simulink model "CLLCResonantConverter"  (R2026a)
settings: Solver=ode23t  StopTime=0.018  FixedStep=1e-4  MaxStep=1e-6  AbsTol=1e-3
PreLoadFcn:
  | % Parameterize the model
  | 
  | if ~exist('CLLCDesign', 'var')
  | CLLCConverterDefaultInputParameters;
  | end
undefined symbols (not defined in the file): CLLCController, CLLCDesign
libraries: fl_lib x46, nesl_utility x45, ee_lib x35, ConverterLibrary x1
(part 1 of 4)
Description:
  | Design of LLC Resonant Converter
settings Model: SimulationMode=accelerator  ExtModeTrigDuration=100  Creator=The MathWorks, Inc.  LastModifiedBy=vsolaise
settings SolverCC: MaxConsecutiveMinStep=10
settings DataIOCC: StateSaveName=tmp_raccel_xout  SignalLoggingName=logsoutCLLCConverter  OutputTimes=[0:1.1*3*Voc/(1*2000):1.1*3*Voc/1]
settings OptimizationCC: EfficientMapNaN2IntZero=off
settings HardwareCC: ProdHWDeviceType=Intel->x86-32 (Windows32)  TargetBitPerPointer=64.0  TargetBitPerSizeT=64.0  TargetBitPerPtrDiffT=64.0  TargetLongLongMode=on  TargetIntDivRoundTo=Zero  TargetEndianess=LittleEndian  TargetWordSize=64.0  TargetHWDeviceType=MATLAB Host  ProdEqTarget=off
settings RTWCC: SystemTargetFile=raccel.tlc  TemplateMakefile=raccel_default_tmf  RTWVerbose=off  RTWUseSimCustomCode=on
settings CodeAppCC: GenerateComments=off  MaxIdLength=128.0  SimulinkBlockComments=off
settings RaccelTargetCC: ExtModeTransport=0.0  ExtModeStaticAllocSize=1000000.0  ENABLE_SLEXEC_SSBRIDGE=1.0  RTWCAPIParams=on  RTWCAPIRootIO=on  MultiwordLength=2048.0
settings SimscapeCC: SimscapeNominalValues="[{\"value\":\"1\",\"unit\":\"A\"},{\"value\":\"1\",\"unit\":\"bar\"},{\"value\":\"1\",\"unit\":\"cm^2\"},{\"value\":\"1\",\"unit\":\"cm^3/s\"},{\"value\":\"1\",\"unit\":\"kJ/kg\"},{\"value\":\"1\",\"unit\":\"kW\"},{\"value\":\"1\",\"unit\":\"l\"},{\"value\":\"1\",\"unit\":\"N\"},{\"value\":\"1\",\"unit\":\"N*m\"},{\"value\":\"1\",\"unit\":\"V\"}]"  SimscapeLogName=SimlogCLLCConverter  SimscapeLogLimitData=off  SimscapeLogDataHistory=5000.0

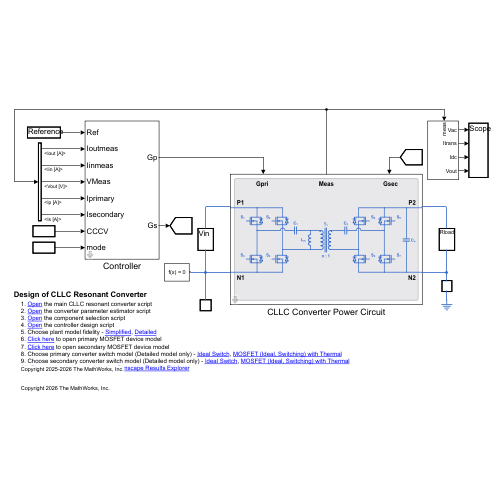
[thumbnail: Simulink's stored preview of the top-level diagram]
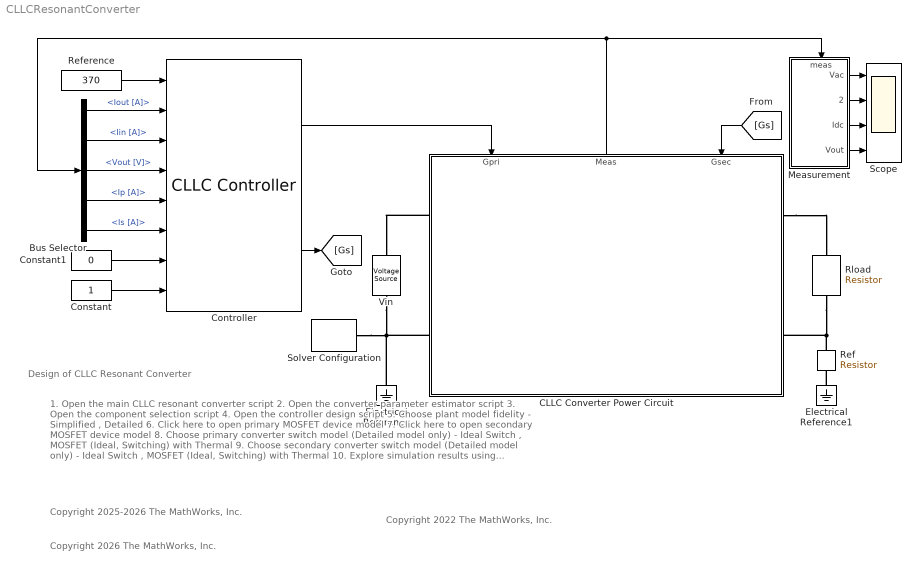
== system CLLCResonantConverter ==
  note: Copyright 2025-2026 The MathWorks, Inc.
  note: 1. Open the main CLLC resonant converter script
      | 2. Open the converter parameter estimator script
      | 3. Open the component selection script
      | 4. Open the controller design script
      | 5. Choose plant model fidelity - Simplified , Detailed
      | 6. Click here to open primary MOSFET device model
      | 7. Click here to open secondary MOSFET device model
      | 8. Choose primary converter switch model (Detailed model only) - Ideal Switch , MOSFET (Ideal, Switching) with Thermal
      | 9. Choose secondary converter switch model (Detailed model only) - Ideal Switch , MOSFET (Ideal, Switching) with Thermal
      | 10. Explore simulation results using Simscape Results Explorer
  note: Design of CLLC Resonant Converter
  note: Copyright 2022 The MathWorks, Inc.
  note: Copyright 2026 The MathWorks, Inc.
  Bus Selector : BusSelector  OutputSignals=Rectifier.Iout [A],Inverter.Iin [A],Rectifier.Vout [V],ResonantTank.Ip [A],ResonantTank.Is [A]
  CLLC Converter Power Circuit : Subsystem  mask(CLLC Converter Plant){modelOption=Simplified, C1=CLLCDesign.C1, C1_unit=F, Rcr1=CLLCDesign.Rcr1, Rcr1_unit=Ohm, C2=CLLCDesign.C2, C2_unit=F, Rcr2=CLLCDesign.Rcr2, Rcr2_unit=Ohm, Llk1=CLLCDesign.Llk1, Llk1_unit=H, R1=CLLCDesign.R1, R1_unit=Ohm, Llk2=CLLCDesign.Llk2, Llk2_unit=H, R2=CLLCDesign.R2, R2_unit=Ohm, Lm=CLLCDesign.Lm, Lm_unit=H, N1=CLLCDesign.N1, N2=CLLCDesign.N2, Co=CLLCDesign.Co, Co_unit=F, Rco=CLLCDesign.Rco, Rco_unit=Ohm, Vco=350, Vco_unit=V, PrimaryDeviceOption=MOSFET (Ideal, Switching) with Thermal, PrimaryRon=0.0001, PrimaryRon_unit=Ohm, PrimaryGoff=1e-5, PrimaryGoff_unit=1/Ohm, PrimaryVth=2.5, PrimaryVth_unit=V, PrimaryVbodydiodeOn=0.6, PrimaryVbodydiodeOn_unit=V, PrimaryRbodydiodeOn=0.0001, PrimaryRbodydiodeOn_unit=Ohm, PrimaryGbodydiodeOff=1e-5, PrimaryGbodydiodeOff_unit=1/Ohm, PrimaryCparasitic=CLLCDesign.Cparasitic, PrimaryCparasitic_unit=F, SecondaryDeviceOption=MOSFET (Ideal, Switching) with Thermal, SecondaryRon=0.0001, SecondaryRon_unit=Ohm, SecondaryGoff=1e-5, SecondaryGoff_unit=1/Ohm, SecondaryVth=2.5, SecondaryVth_unit=V, SecondaryVbodydiodeOn=0.6, SecondaryVbodydiodeOn_unit=V, SecondaryRbodydiodeOn=0.0001, SecondaryRbodydiodeOn_unit=Ohm, SecondaryGbodydiodeOff=1e-5, SecondaryGbodydiodeOff_unit=1/Ohm, SecondaryCparasitic=CLLCDesign.Cparasitic, SecondaryCparasitic_unit=F, PrimarySimTemp=25, PrimarySimTemp_unit=degC, SecondarySimTemp=25, SecondarySimTemp_unit=degC}
      mask prompts: modelOption "Model option"; C1 "Primary resonant capacitance (C1)"; Rcr1 "Primary resonant capacitor ESR (Rcr1)"; C2 "Secondary resonant capacitance (C2)"; Rcr2 "Secondary resonant capacitor ESR (Rcr2)"; Llk1 "Primary leakage inductance (Llk1)"; R1 "Primary resistance (R1)"; Llk2 "Secondary leakage inductance (Llk2)"; R2 "Secondary resistance (R2)"; Lm "Magnetizing inductance (Lm)"; N1 "Transformer primary number of turns (N1)"; N2 "Transformer secondary number of turns (N2)"; Co "Secondary output capacitance (Co)"; Rco "Secondary output capacitance ESR (Rco)"; Vco "Initial output capacitor voltage"; PrimaryDeviceOption "Select the primary switching device"; PrimaryRon "On-state resistance"; PrimaryGoff "Off-state conductance"; PrimaryVth "Threshold voltage"; PrimaryVbodydiodeOn "Body diode forward voltage"; PrimaryRbodydiodeOn "Body diode on-resistance"; PrimaryGbodydiodeOff "Body diode off-conductance"; PrimaryCparasitic "MOSFET parasitic capacitance"; SecondaryDeviceOption "Select the secondary switching device"; SecondaryRon "On-state resistance"; SecondaryGoff "Off-state conductance"; SecondaryVth "Threshold voltage"; SecondaryVbodydiodeOn "Body diode forward voltage"; SecondaryRbodydiodeOn "Body diode on-resistance"; SecondaryGbodydiodeOff "Body diode off-conductance"; SecondaryCparasitic "MOSFET parasitic capacitance"; PrimarySimTemp "Simulation temperature"; SecondarySimTemp "Simulation temperature"
      mask help: This block models the power circuit of the CLLC resonant converter. You can choose between different semicondcutor switch model for primary and secondaryconverter. You can choose between ideal semiconductor switch, MOSFET without thermal port and tabulated MOSFET with thermal port.
      mask init:
      | %% Unit conversion: convert displayed values to base SI units
      | convMap = containers.Map( ...
      |     {'W','kW','MW','V','kV','mV','F','mF','uF','nF','pF', ...
      |      'H','mH','uH','nH','Ohm','kOhm','mOhm','S','mS','1/Ohm'}, ...
      |     {1, 1e3, 1e6, 1, 1e3, 1e-3, 1, 1e-3, 1e-6, 1e-9, 1e-12, ...
      |      1, 1e-3, 1e-6, 1e-9, 1, 1e3, 1e-3, 1, 1e-3, 1});
      | C1 = C1 * convMap(C1_unit);
      | Rcr1 = Rcr1 * convMap(Rcr1_unit);
      | C2 = C2 * convMap(C2_unit);
      | Rcr2 = Rcr2 * convMap(Rcr2_unit);
      | Llk1 = Llk1 * convMap(Llk1_unit);
      | R1 = R1 * convMap(R1_unit);
      | Llk2 = Llk2 * convMap(Llk2_unit);
      | R2 = R2 * convMap(R2_unit);
      | Lm = Lm * convMap(Lm_unit);
      | Co = Co * convMap(Co_unit);
      | Rco = Rco * convMap(Rco_unit);
      | Vco = Vco * convMap(Vco_unit);
      | PrimaryRon = PrimaryRon * convMap(PrimaryRon_unit);
      | PrimaryGoff = PrimaryGoff * convMap(PrimaryGoff_unit);
      | PrimaryVth = PrimaryVth * convMap(PrimaryVth_unit);
      | PrimaryVbodydiodeOn = PrimaryVbodydiodeOn * convMap(PrimaryVbodydiodeOn_unit);
      | PrimaryRbodydiodeOn = PrimaryRbodydiodeOn * convMap(PrimaryRbodydiodeOn_unit);
      | PrimaryGbodydiodeOff = PrimaryGbodydiodeOff * convMap(PrimaryGbodydiodeOff_unit);
      | PrimaryCparasitic = PrimaryCparasitic * convMap(PrimaryCparasitic_unit);
      | SecondaryRon = SecondaryRon * convMap(SecondaryRon_unit);
      | SecondaryGoff = SecondaryGoff * convMap(SecondaryGoff_unit);
      | SecondaryVth = SecondaryVth * convMap(SecondaryVth_unit);
      | SecondaryVbodydiodeOn = SecondaryVbodydiodeOn * convMap(SecondaryVbodydiodeOn_unit);
      | SecondaryRbodydiodeOn = SecondaryRbodydiodeOn * convMap(SecondaryRbodydiodeOn_unit);
      | SecondaryGbodydiodeOff = SecondaryGbodydiodeOff * convMap(SecondaryGbodydiodeOff_unit);
      | SecondaryCparasitic = SecondaryCparasitic * convMap(SecondaryCparasitic_unit);
      | % Simulation temperature (primary bridge, thermal MOSFETs)
      | % Temperature is an OFFSET unit (K = degC + 273.15), so it cannot use the
      | % multiplicative convMap above; convert it explicitly. PrimarySimTemp_K is read directly
      | % by each primary thermal MOSFET junction-temperature initial target and by every
      | % Temperature Source in the primary bridge.
      | if strcmp(PrimarySimTemp_unit, 'degC')
      |     PrimarySimTemp_K = PrimarySimTemp + 273.15;
      | elseif strcmp(PrimarySimTemp_unit, 'K')
      |     PrimarySimTemp_K = PrimarySimTemp;
      | else
      |     error('CLLC Converter Power Circuit: unrecognized simulation-temperature unit "%s" (expected degC or K).', PrimarySimTemp_unit);
      | end
      | % Simulation temperature (secondary bridge, thermal MOSFETs)
      | % Temperature is an OFFSET unit (K = degC + 273.15), so it cannot use the
      | % multiplicative convMap above; convert it explicitly. SecondarySimTemp_K is read directly
      | % by each secondary thermal MOSFET junction-temperature initial target and by every
      | % Temperature Source in the secondary bridge.
      | if strcmp(SecondarySimTemp_unit, 'degC')
      |     SecondarySimTemp_K = SecondarySimTemp + 273.15;
      | elseif strcmp(SecondarySimTemp_unit, 'K')
      |     SecondarySimTemp_K = SecondarySimTemp;
      | else
      |     error('CLLC Converter Power Circuit: unrecognized simulation-temperature unit "%s" (expected degC or K).', SecondarySimTemp_unit);
      | end
      settings: CopyFcn="set_param(gcbh,\"LinkStatus\",\"none\");"  PortSchema="{\"entries\":[{\"content\":{\"sides\":[{\"content\":{\"connectorIds\":[\"LConn1\",\"LConn2\"]},\"type\":\"ConnectorPlacement.EquallySpacedRectSide\",\"uuid\":\"0e984043-8111-4613-9feb-f4d4d19f792a\"},{\"content\":{\"connectorIds\":[\"RConn1\",\"RConn2\"],\"side\":\"RIGHT\"},\"type\":\"ConnectorPlacement.EquallySpacedRectSide\",\"uuid\":\"aee9207a-aaf7-4114-a348-153041cb19a5\"},{\"content\":{\"connectorIds\":[\"In1\",\"Out1\",\"In2\"],\"side\":\"TOP\"},\"type\":\"ConnectorPlacement.EquallySpacedRectSide\",\"uuid\":\"cf17a722-cb18-4642-bf19-4f4ee8ce3a25\"}]},\"type\":\"ConnectorPlacement.EquallySpacedConnector\",\"uuid\":\"0a50e5d5-a4bf-4817-9816-42fb9bad860d\"}],\"packageUris\":[\"http://schema.mathworks.com/mf0/Connector/R2020b\"],\"version\":\"1.0\"}"
      mask Help: web('CLLCPowerCircuit.html')
      mask TypeOptions modelOption: Simplified | Detailed
      mask Callback modelOption: selectCLLCConverterModelOption(gcb);
      mask TypeOptions C1_unit: F | mF | uF | nF | pF
      mask TypeOptions Rcr1_unit: Ohm | kOhm | mOhm
      mask TypeOptions C2_unit: F | mF | uF | nF | pF
      mask TypeOptions Rcr2_unit: Ohm | kOhm | mOhm
      mask TypeOptions Llk1_unit: H | mH | uH | nH
      mask TypeOptions R1_unit: Ohm | kOhm | mOhm
      mask TypeOptions Llk2_unit: H | mH | uH | nH
      mask TypeOptions R2_unit: Ohm | kOhm | mOhm
      mask TypeOptions Lm_unit: H | mH | uH | nH
      mask TypeOptions Co_unit: F | mF | uF | nF | pF
      mask TypeOptions Rco_unit: Ohm | kOhm | mOhm
      mask TypeOptions Vco_unit: V | kV | mV
      mask TypeOptions PrimaryDeviceOption: Ideal Switch | MOSFET (Ideal, Switching) with Thermal
      mask Callback PrimaryDeviceOption: selectCLLCPrimaryMOSFET(gcb);
      mask TypeOptions PrimaryRon_unit: Ohm | kOhm | mOhm
      mask TypeOptions PrimaryGoff_unit: 1/Ohm | S | mS
      mask TypeOptions PrimaryVth_unit: V | kV | mV
      mask TypeOptions PrimaryVbodydiodeOn_unit: V | mV
      mask TypeOptions PrimaryRbodydiodeOn_unit: Ohm | kOhm | mOhm
      mask TypeOptions PrimaryGbodydiodeOff_unit: 1/Ohm | S | mS
      mask TypeOptions PrimaryCparasitic_unit: F | mF | uF | nF | pF
      mask TypeOptions SecondaryDeviceOption: Ideal Switch | MOSFET (Ideal, Switching) with Thermal
      mask Callback SecondaryDeviceOption: selectCLLCSecondaryMOSFET(gcb);
      mask TypeOptions SecondaryRon_unit: Ohm | kOhm | mOhm
      mask TypeOptions SecondaryGoff_unit: 1/Ohm | S | mS
      mask TypeOptions SecondaryVth_unit: V | kV | mV
      mask TypeOptions SecondaryVbodydiodeOn_unit: V | mV
      mask TypeOptions SecondaryRbodydiodeOn_unit: Ohm | kOhm | mOhm
      mask TypeOptions SecondaryGbodydiodeOff_unit: 1/Ohm | S | mS
      mask TypeOptions SecondaryCparasitic_unit: F | mF | uF | nF | pF
      mask TypeOptions PrimarySimTemp_unit: degC | K
      mask TypeOptions SecondarySimTemp_unit: degC | K
      mask DialogControl ParameterGroupVar Prompt: CLLC Resonant Converter Plant
      mask DialogControl CLLCTank Prompt: CLLC converter parameters
      mask DialogControl TransformerParameters Prompt: Transformer
      mask DialogControl PrimarySwitch Prompt: Primary semiconductor switch
      mask DialogControl PrimaryOpenMOSFETMask Prompt: Open the MOSFET block mask
      mask DialogControl PrimaryOpenMOSFETMask Callback: openCLLCDeviceMask(gcb, 'primaryThermalMOSFET');
      mask DialogControl PrimaryApplyMOSFETParam Prompt: Apply parameters to all primary MOSFET blocks
      mask DialogControl PrimaryApplyMOSFETParam Callback: applyCLLCDeviceParameters(gcb, 'primaryThermalMOSFET');
      mask DialogControl SecondarySwitch Prompt: Secondary semiconductor switch
      mask DialogControl SecondaryOpenMOSFETMask Prompt: Open the MOSFET block mask
      mask DialogControl SecondaryOpenMOSFETMask Callback: openCLLCDeviceMask(gcb, 'secondaryThermalMOSFET');
      mask DialogControl SecondaryApplyMOSFETParam Prompt: Apply parameters to all secondary MOSFET blocks
      mask DialogControl SecondaryApplyMOSFETParam Callback: applyCLLCDeviceParameters(gcb, 'secondaryThermalMOSFET');
      mask DialogControl ExportPanel Prompt: Export to Unmasked Subsystem
      mask DialogControl ExportInfo Prompt: To customize the converter, export it as an unmasked subsystem with the active variant flattened - a standalone, fully-editable circuit plus a parameter file. Requires the "Variant Manager for Simulink" add-on.
      mask DialogControl exportToModel Prompt: Export
      mask DialogControl exportToModel Callback: exportConverterModelFromMask(gcb);
      mask Display: image('CLLCConverterIcon.svg');
  Constant : Constant
  Constant1 : Constant  Value=0
  Controller : ConverterLibrary/Controller/Soft-Switching Converters/CLLC Controller  controllerDomain=Continuous  resFreq=CLLCDesign.resonantFreq  ratedPower=CLLCSpec.ratedOutputPower.value  Fmin=CLLCController.minPUfrequency  Fmax=CLLCController.maxPUfrequency  Tdead=CLLCController.deadTime  VdcValue=CLLCSpec.maxInputVoltage.value  Kpv=CLLCController.Kpv  Kiv=CLLCController.Kiv  Kid=0  IdcMax=2.5  IdcMin=-2.5  cntrlSelect=2P2Z compensator  Kc=CLLCCompensator.Ki  numSdomain=CLLCCompensator.numSDomain  denSdomain=CLLCCompensator.denSDomain  numZdomain=CLLCCompensator.numZDomain  denZdomain=CLLCCompensator.denZDomain  Kp=CLLCController.Kp  Ki=CLLCController.Ki  Ith=CLLCCompensator.SRCurrentThreshold  Ibw=300000  vcoSelect=Constant rate  vcoGain=CLLCController.constantVCOGain  vcoGainVec=CLLCController.vcoGainVec  pwmSampleTime=CLLCController.deadTime/2  TsVoltage=CLLCController.TsVoltage  TsCurrent=CLLCController.TsCurrent
      link override 2P2Z Compensator: LabelModeActiveChoice=SCompensator
      link override VCO: LabelModeActiveChoice=Constant
      settings: SourceProductName=Simscape Power Converter Components
  Electrical Reference : fl_lib/Electrical/Electrical Elements/Electrical Reference
  Electrical Reference1 : fl_lib/Electrical/Electrical Elements/Electrical Reference
  Measurement : Subsystem
      settings: PortSchema="{\"entries\":[{\"content\":{\"sides\":[{\"content\":{},\"type\":\"ConnectorPlacement.EquallySpacedRectSide\",\"uuid\":\"b5c92219-bd3b-44a8-8a16-1ea587978409\"},{\"content\":{\"connectorIds\":[\"Out1\",\"Out2\",\"Out3\",\"Out4\"],\"side\":\"RIGHT\"},\"type\":\"ConnectorPlacement.EquallySpacedRectSide\",\"uuid\":\"b58951fa-0a4a-415c-91fc-a01c5851cf7b\"},{\"content\":{\"connectorIds\":[\"In1\"],\"side\":\"TOP\"},\"type\":\"ConnectorPlacement.EquallySpacedRectSide\",\"uuid\":\"5d7f8742-bb02-4261-b191-4137e05aff11\"}]},\"type\":\"ConnectorPlacement.EquallySpacedConnector\",\"uuid\":\"cec0d984-b283-4d36-85e7-6ccc2789e1e2\"}],\"packageUris\":[\"http://schema.mathworks.com/mf0/Connector/R2020b\"],\"version\":\"1.0\"}"
  Ref : fl_lib/Electrical/Electrical Elements/Resistor  R=1e5 Ohm  i_specify=off  i_priority=None  i=0 A  i_nominal_specify=off  i_nominal_value=1  i_nominal_unit=A  v_specify=off  v_priority=None  v=0 V  v_nominal_specify=off  v_nominal_value=1  v_nominal_unit=V
  Reference : Constant  Value=370
  Rload : fl_lib/Electrical/Electrical Elements/Resistor  R=19.55 Ohm  i_specify=off  i_priority=None  i=0 A  i_nominal_specify=off  i_nominal_value=1  i_nominal_unit=A  v_specify=off  v_priority=None  v=0 V  v_nominal_specify=off  v_nominal_value=1  v_nominal_unit=V
  Scope : Scope  NumInputPorts=4
      settings: Title=Resonant Tank Voltages  ActiveDisplayYMinimum=-489.00804394108224  ActiveDisplayYMaximum=489.00846158085653
  Solver Configuration : nesl_utility/Solver Configuration  PhysicalDomain=network_engine_domain  SubClassName=solver  LeftPortType=input  RightPortType=generic  Tones=[]  Harmonics=[]  SimulateNoise=off  Profile=off  UseLocalSampling=off  EnableSwitchedLinearOptims=on  FrequencyDomain=off  UseCCode=off  RelTol=0.001  AbsTol=0.001  MinStep=1e-09  ToWorkspace=off  RevertToSquareIcSolve=off  NumHomotopyIterations=100  PhasorMode=off  PhasorModeNumHarmonics=1  ConsistencySolver=NEWTON_XTOL_AFTER_FTOL  CanonicalOrdering=UNORDERED  OptimizeIntermediates=UNOPTIMIZED  IndexReductionMethod=DerivativeReplacement  DoDC=off  ResidualTolerance=1e-09  ConsistencyTolSource=GLOBAL  ConsistencyAbsTol=0.001  ConsistencyRelTol=0.001  ConsistencyTolFactor=0.001  UseLocalSolver=on  LocalSolverChoice=NE_BACKWARD_EULER_ADVANCER  ResolveIndetEquations=off  FunctionEvalNumThread=1  LocalSolverSampleTime=CLLCController.deadTime/3  DoFixedCost=on  MaxNonlinIter=5  MaxModeIter=10  ComputeImpulses=off  ImpulseIterations=2  LinearAlgebra=auto  LinearAlgebraNumThread=0  EquationFormulation=NE_TIME_EF  DelaysMemoryBudget=1024  AutomaticFiltering=on  FilteringTimeConstant=0.001  PartitionStorageMethod=AS_NEEDED  PartitionMemoryBudget=1024  PartitionMethod=ROBUST  MultibodyUseLocalSolver=off  MultibodyLocalSolverChoice=ODE1  MultibodyLocalSolverSampleTime=0.001
  Vin : ee_lib/Sources/Voltage Source  dc_voltage=390 V  ac_voltage=0 V  ac_shift=0 rad  ac_frequency=0 Hz  noise_mode=ee.enum.sources.noise.Disabled  PSD=0 V^2/Hz  sample_time=1e-3 s  repeatability=ee.enum.sources.repeatability.NotRepeatable  user_seed=0  auto_seed=3499211588  i_specify=off  i_priority=None  i=0 A  i_nominal_specify=off  i_nominal_value=1  i_nominal_unit=A  v_specify=off  v_priority=None  v=0 V  v_nominal_specify=off  v_nominal_value=1  v_nominal_unit=V
  wires:
  Measurement/1(Vac) -> Scope/1
  Measurement/2(Itrans) -> Scope/2
  Measurement/3(Idc) -> Scope/3
  Measurement/4(Vout) -> Scope/4
  Controller/2 -> [Gs]
  Controller/1 -> CLLC Converter Power Circuit/1(Gpri)
  [Gs] -> CLLC Converter Power Circuit/2(Gsec)
  Bus Selector/5 -> Controller/6  "<Is [A]>"
  Bus Selector/4 -> Controller/5  "<Ip [A]>"
  Constant1/1 -> Controller/7
  CLLC Converter Power Circuit/1(Meas) -> Measurement/1(meas), Bus Selector/1
  Bus Selector/1 -> Controller/2  "<Iout [A]>"
  Bus Selector/2 -> Controller/3  "<Iin [A]>"
  Bus Selector/3 -> Controller/4  "<Vout [V]>"
  Reference/1 -> Controller/1
  Constant/1 -> Controller/8
  connections:
  Vin/RConn1 -- Solver Configuration/RConn1 -- Electrical Reference/LConn1 -- CLLC Converter Power Circuit/LConn2
  Electrical Reference1/LConn1 -- Ref/RConn1
  CLLC Converter Power Circuit/LConn1 -- Vin/LConn1
  CLLC Converter Power Circuit/RConn1 -- Rload/LConn1
  Ref/LConn1 -- Rload/RConn1 -- CLLC Converter Power Circuit/RConn2

== system CLLCResonantConverter/CLLC Converter Power Circuit ==
  Gpri : Inport
  Gsec : Inport  Port=2
  CLLCConverterVariant : Subsystem  Variant=on  VariantControlMode=label  LabelModeActiveChoice=SimplifiedModel
  P1 : PMIOPort  Side=Left
  N1 : PMIOPort  Port=2  Side=Left
  P2 : PMIOPort  Port=3  Side=Right
  N2 : PMIOPort  Port=4  Side=Right
  Meas : Outport
  wires:
  CLLCConverterVariant/1(Meas) -> Meas/1
  Gsec/1 -> CLLCConverterVariant/2(Gsec)
  Gpri/1 -> CLLCConverterVariant/1(Gpri)
  connections:
  CLLCConverterVariant/RConn2 -- N2/RConn1
  CLLCConverterVariant/RConn1 -- P2/RConn1
  CLLCConverterVariant/LConn2 -- N1/RConn1
  CLLCConverterVariant/LConn1 -- P1/RConn1

== system CLLCResonantConverter/Measurement ==
  BusElementIn5 : Inport  PortName=meas  Element=ResonantTank.Vp [V]
  BusElementIn6 : Inport  PortName=meas  Element=ResonantTank.Ip [A]
  BusElementIn7 : Inport  PortName=meas  Element=ResonantTank.Is [A]
  BusElementIn8 : Inport  PortName=meas  Element=ResonantTank.Vs [A]
  BusElementIn10 : Inport  PortName=meas  Element=Inverter.Iin [A]
  BusElementIn9 : Inport  PortName=meas  Element=Rectifier.Iout [A]
  BusElementIn : Inport  PortName=meas  Element=Rectifier.Vout [V]
  Bus Creator : BusCreator  Inputs=2
  Bus Creator1 : BusCreator  Inputs=2
  Bus Creator2 : BusCreator  Inputs=2
  Vac : Outport
  Itrans : Outport  Port=2
  Idc : Outport  Port=3
  Vout : Outport  Port=4
  wires:
  BusElementIn5/1 -> Bus Creator/1  "Vprimary"
  BusElementIn8/1 -> Bus Creator/2  "Vsecondary"
  BusElementIn10/1 -> Bus Creator2/2  "Iin"
  BusElementIn/1 -> Vout/1  "Vout"
  Bus Creator/1 -> Vac/1
  BusElementIn9/1 -> Bus Creator2/1  "Iout"
  Bus Creator2/1 -> Idc/1
  BusElementIn6/1 -> Bus Creator1/1  "Iprimary"
  BusElementIn7/1 -> Bus Creator1/2  "Isecondary"
  Bus Creator1/1 -> Itrans/1

== system CLLCResonantConverter/CLLC Converter Power Circuit/CLLCConverterVariant ==
  Gpri : Inport
  Gsec : Inport  Port=2
  DetailedModel : Subsystem  VariantControl=DetailedModel
  SimplifiedModel : Subsystem  VariantControl=SimplifiedModel
  P1 : PMIOPort  Side=Left
  P2 : PMIOPort  Port=2  Side=Right
  N1 : PMIOPort  Port=3  Side=Left
  N2 : PMIOPort  Port=4  Side=Right
  Meas : Outport

== system CLLCResonantConverter/CLLC Converter Power Circuit/CLLCConverterVariant/DetailedModel ==
  Gpri : Inport
  Gsec : Inport  Port=2
  Bus Creator : BusCreator  Inputs=3
  Primary Converter : Subsystem
      settings: PortSchema="{\"entries\":[{\"content\":{\"sides\":[{\"content\":{\"connectorIds\":[\"LConn1\",\"LConn2\"]},\"type\":\"ConnectorPlacement.EquallySpacedRectSide\",\"uuid\":\"5f98eff0-54e4-47a8-aeeb-0279cba14f26\"},{\"content\":{\"connectorIds\":[\"RConn1\",\"RConn2\"],\"side\":\"RIGHT\"},\"type\":\"ConnectorPlacement.EquallySpacedRectSide\",\"uuid\":\"71acbbb6-1fc8-426c-b389-5d494eb18bfd\"},{\"content\":{\"connectorIds\":[\"In1\",\"Out1\"],\"side\":\"TOP\"},\"type\":\"ConnectorPlacement.EquallySpacedRectSide\",\"uuid\":\"dc77ee05-1f57-4323-bfda-b0076e2d1ee5\"}]},\"type\":\"ConnectorPlacement.EquallySpacedConnector\",\"uuid\":\"8d0b8c05-d5c5-4033-af60-ebdb639bdc40\"}],\"packageUris\":[\"http://schema.mathworks.com/mf0/Connector/R2020b\"],\"version\":\"1.0\"}"
  Resonant Tank : Subsystem
      settings: PortSchema="{\"entries\":[{\"content\":{\"sides\":[{\"content\":{\"connectorIds\":[\"LConn1\",\"LConn2\"]},\"type\":\"ConnectorPlacement.EquallySpacedRectSide\",\"uuid\":\"d505f362-3b8e-4dee-9b5b-731d75550efb\"},{\"content\":{\"connectorIds\":[\"RConn1\",\"RConn2\"],\"side\":\"RIGHT\"},\"type\":\"ConnectorPlacement.EquallySpacedRectSide\",\"uuid\":\"66ab4b84-9b7a-404b-b3f6-3ac1c371ea42\"},{\"content\":{\"connectorIds\":[\"Out1\"],\"side\":\"TOP\"},\"type\":\"ConnectorPlacement.EquallySpacedRectSide\",\"uuid\":\"00605859-d490-4a3b-aace-391362dfba7e\"}]},\"type\":\"ConnectorPlacement.EquallySpacedConnector\",\"uuid\":\"a210fe68-7181-499f-8e1c-ccfe71b42a4c\"}],\"packageUris\":[\"http://schema.mathworks.com/mf0/Connector/R2020b\"],\"version\":\"1.0\"}"
      mask Display: image('CLLCTransformerIcon.png');
  Secondary Converter : Subsystem
      settings: PortSchema="{\"entries\":[{\"content\":{\"sides\":[{\"content\":{\"connectorIds\":[\"LConn1\",\"LConn2\"]},\"type\":\"ConnectorPlacement.EquallySpacedRectSide\",\"uuid\":\"4786b3cc-2245-4c72-a50b-9c63e4ad3d8a\"},{\"content\":{\"connectorIds\":[\"RConn1\",\"RConn2\"],\"side\":\"RIGHT\"},\"type\":\"ConnectorPlacement.EquallySpacedRectSide\",\"uuid\":\"250a01d0-bf95-4e01-bf69-d866bcf3b7bd\"},{\"content\":{\"connectorIds\":[\"In1\",\"Out1\"],\"side\":\"TOP\"},\"type\":\"ConnectorPlacement.EquallySpacedRectSide\",\"uuid\":\"52730d18-084b-4644-8b2a-b54c84fa88ec\"}]},\"type\":\"ConnectorPlacement.EquallySpacedConnector\",\"uuid\":\"d24cae2a-f132-4f5a-ac35-d7440d7a99e9\"}],\"packageUris\":[\"http://schema.mathworks.com/mf0/Connector/R2020b\"],\"version\":\"1.0\"}"
  P1 : PMIOPort  Side=Left
  P2 : PMIOPort  Port=2  Side=Right
  N1 : PMIOPort  Port=3  Side=Left
  N2 : PMIOPort  Port=4  Side=Right
  Meas : Outport
  wires:
  Gpri/1 -> Primary Converter/1(G)
  Gsec/1 -> Secondary Converter/1(G)
  Primary Converter/1(meas) -> Bus Creator/1  "Inverter"
  Secondary Converter/1(meas) -> Bus Creator/3  "Rectifier"
  Bus Creator/1 -> Meas/1
  Resonant Tank/1(meas) -> Bus Creator/2  "ResonantTank"
  connections:
  N1/RConn1 -- Primary Converter/LConn2
  N2/RConn1 -- Secondary Converter/RConn2
  Resonant Tank/LConn1 -- Primary Converter/RConn1
  Resonant Tank/RConn2 -- Secondary Converter/LConn2
  P1/RConn1 -- Primary Converter/LConn1
  P2/RConn1 -- Secondary Converter/RConn1
  Resonant Tank/LConn2 -- Primary Converter/RConn2
  Resonant Tank/RConn1 -- Secondary Converter/LConn1

== system CLLCResonantConverter/CLLC Converter Power Circuit/CLLCConverterVariant/SimplifiedModel ==
  Gpri : Inport
  Gsec : Inport  Port=2
  Bus Creator : BusCreator  Inputs=3
  Primary Converter : Subsystem
      settings: PortSchema="{\"entries\":[{\"content\":{\"sides\":[{\"content\":{\"connectorIds\":[\"LConn1\",\"LConn2\"]},\"type\":\"ConnectorPlacement.EquallySpacedRectSide\",\"uuid\":\"5f98eff0-54e4-47a8-aeeb-0279cba14f26\"},{\"content\":{\"connectorIds\":[\"RConn1\",\"RConn2\"],\"side\":\"RIGHT\"},\"type\":\"ConnectorPlacement.EquallySpacedRectSide\",\"uuid\":\"71acbbb6-1fc8-426c-b389-5d494eb18bfd\"},{\"content\":{\"connectorIds\":[\"In1\",\"Out1\"],\"side\":\"TOP\"},\"type\":\"ConnectorPlacement.EquallySpacedRectSide\",\"uuid\":\"dc77ee05-1f57-4323-bfda-b0076e2d1ee5\"}]},\"type\":\"ConnectorPlacement.EquallySpacedConnector\",\"uuid\":\"8d0b8c05-d5c5-4033-af60-ebdb639bdc40\"}],\"packageUris\":[\"http://schema.mathworks.com/mf0/Connector/R2020b\"],\"version\":\"1.0\"}"
  Resonant Tank : Subsystem
      settings: PortSchema="{\"entries\":[{\"content\":{\"sides\":[{\"content\":{\"connectorIds\":[\"LConn1\",\"LConn2\"]},\"type\":\"ConnectorPlacement.EquallySpacedRectSide\",\"uuid\":\"d505f362-3b8e-4dee-9b5b-731d75550efb\"},{\"content\":{\"connectorIds\":[\"RConn1\",\"RConn2\"],\"side\":\"RIGHT\"},\"type\":\"ConnectorPlacement.EquallySpacedRectSide\",\"uuid\":\"66ab4b84-9b7a-404b-b3f6-3ac1c371ea42\"},{\"content\":{\"connectorIds\":[\"Out1\"],\"side\":\"TOP\"},\"type\":\"ConnectorPlacement.EquallySpacedRectSide\",\"uuid\":\"00605859-d490-4a3b-aace-391362dfba7e\"}]},\"type\":\"ConnectorPlacement.EquallySpacedConnector\",\"uuid\":\"a210fe68-7181-499f-8e1c-ccfe71b42a4c\"}],\"packageUris\":[\"http://schema.mathworks.com/mf0/Connector/R2020b\"],\"version\":\"1.0\"}"
      mask Display: image('CLLCTransformerIcon.png')
  Secondary Converter : Subsystem
      settings: PortSchema="{\"entries\":[{\"content\":{\"sides\":[{\"content\":{\"connectorIds\":[\"LConn1\",\"LConn2\"]},\"type\":\"ConnectorPlacement.EquallySpacedRectSide\",\"uuid\":\"4786b3cc-2245-4c72-a50b-9c63e4ad3d8a\"},{\"content\":{\"connectorIds\":[\"RConn1\",\"RConn2\"],\"side\":\"RIGHT\"},\"type\":\"ConnectorPlacement.EquallySpacedRectSide\",\"uuid\":\"250a01d0-bf95-4e01-bf69-d866bcf3b7bd\"},{\"content\":{\"connectorIds\":[\"In1\",\"Out1\"],\"side\":\"TOP\"},\"type\":\"ConnectorPlacement.EquallySpacedRectSide\",\"uuid\":\"52730d18-084b-4644-8b2a-b54c84fa88ec\"}]},\"type\":\"ConnectorPlacement.EquallySpacedConnector\",\"uuid\":\"d24cae2a-f132-4f5a-ac35-d7440d7a99e9\"}],\"packageUris\":[\"http://schema.mathworks.com/mf0/Connector/R2020b\"],\"version\":\"1.0\"}"
  P1 : PMIOPort  Side=Left
  P2 : PMIOPort  Port=2  Side=Right
  N1 : PMIOPort  Port=3  Side=Left
  N2 : PMIOPort  Port=4  Side=Right
  Meas : Outport
  wires:
  Resonant Tank/1(meas) -> Bus Creator/2  "ResonantTank"
  Bus Creator/1 -> Meas/1
  Secondary Converter/1(meas) -> Bus Creator/3  "Rectifier"
  Primary Converter/1(meas) -> Bus Creator/1  "Inverter"
  Gsec/1 -> Secondary Converter/1(G)
  Gpri/1 -> Primary Converter/1(G)
  connections:
  Resonant Tank/RConn1 -- Secondary Converter/LConn1
  Resonant Tank/LConn2 -- Primary Converter/RConn2
  P2/RConn1 -- Secondary Converter/RConn1
  P1/RConn1 -- Primary Converter/LConn1
  Resonant Tank/RConn2 -- Secondary Converter/LConn2
  Resonant Tank/LConn1 -- Primary Converter/RConn1
  N2/RConn1 -- Secondary Converter/RConn2
  N1/RConn1 -- Primary Converter/LConn2

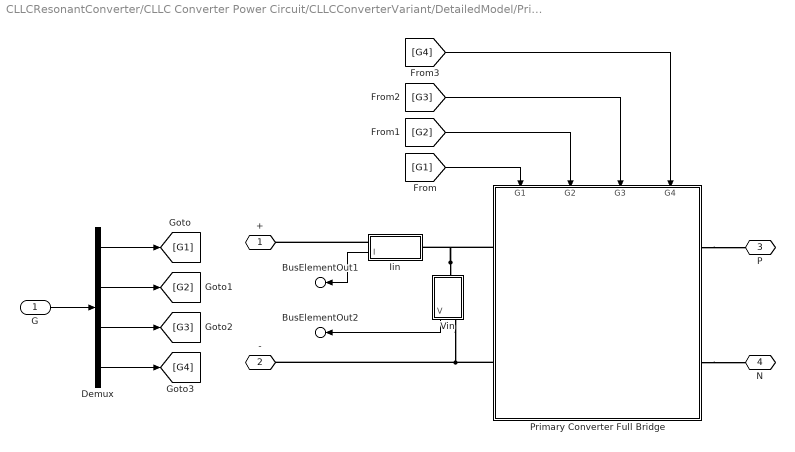
== system CLLCResonantConverter/CLLC Converter Power Circuit/CLLCConverterVariant/DetailedModel/Primary Converter ==
  G : Inport
  Demux : Demux
  Iin : Subsystem
      settings: PortSchema="{\"entries\":[{\"content\":{\"sides\":[{\"content\":{\"connectorIds\":[\"LConn1\",\"Out1\"]},\"type\":\"ConnectorPlacement.EquallySpacedRectSide\",\"uuid\":\"e749c2ff-fd60-426f-a769-b61a7dfe80d2\"},{\"content\":{\"connectorIds\":[\"RConn1\"],\"side\":\"RIGHT\"},\"type\":\"ConnectorPlacement.EquallySpacedRectSide\",\"uuid\":\"f3bb02bd-f8d2-4326-b68c-6f969fa4ac22\"},{\"content\":{\"side\":\"TOP\"},\"type\":\"ConnectorPlacement.EquallySpacedRectSide\",\"uuid\":\"9ab7a0d1-20d8-49e4-8eb3-54d34434204c\"}]},\"type\":\"ConnectorPlacement.EquallySpacedConnector\",\"uuid\":\"19e2a6d5-13f4-47de-bb59-b826817cba83\"}],\"packageUris\":[\"http://schema.mathworks.com/mf0/Connector/R2020b\"],\"version\":\"1.0\"}"
      mask Display: disp("I")
  Primary Converter Full Bridge : Subsystem  Variant=on  VariantControlMode=label  LabelModeActiveChoice=IdealMOSFETwithThermal
      settings: PortSchema="{\"entries\":[{\"content\":{\"sides\":[{\"content\":{\"connectorIds\":[\"LConn1\",\"LConn2\"]},\"type\":\"ConnectorPlacement.EquallySpacedRectSide\",\"uuid\":\"27c41940-d662-4779-afdd-48b642f77411\"},{\"content\":{\"connectorIds\":[\"RConn1\",\"RConn2\"],\"side\":\"RIGHT\"},\"type\":\"ConnectorPlacement.EquallySpacedRectSide\",\"uuid\":\"b0072b01-add1-4b0f-b94e-e1b6c9886b0e\"},{\"content\":{\"connectorIds\":[\"In1\",\"In2\",\"In3\",\"In4\"],\"side\":\"TOP\"},\"type\":\"ConnectorPlacement.EquallySpacedRectSide\",\"uuid\":\"c43bed80-422d-49db-9596-8b38d5c3e411\"},{\"content\":{\"side\":\"BOTTOM\"},\"type\":\"ConnectorPlacement.EquallySpacedRectSide\",\"uuid\":\"01f06046-f57e-45b0-bca5-368a5a543f97\"}]},\"type\":\"ConnectorPlacement.EquallySpacedConnector\",\"uuid\":\"2fcb5370-6bd7-4702-bf87-ebedbb7e376c\"}],\"packageUris\":[\"http://schema.mathworks.com/mf0/Connector/R2020b\"],\"version\":\"1.0\"}"
  Vin : Subsystem
      mask Display: disp("V")
  + : PMIOPort  Side=Left
  - : PMIOPort  Port=2  Side=Left
  P : PMIOPort  Port=3  Side=Right
  N : PMIOPort  Port=4  Side=Right
  BusElementOut2 : Outport  PortName=meas  Element=Vin [V]
  BusElementOut1 : Outport  PortName=meas  Element=Iin [A]
  wires:
  Iin/1(I) -> BusElementOut1/1
  Vin/1(V) -> BusElementOut2/1
  Demux/4 -> [G4]
  Demux/3 -> [G3]
  Demux/2 -> [G2]
  Demux/1 -> [G1]
  G/1 -> Demux/1
  [G1] -> Primary Converter Full Bridge/1(G1)
  [G2] -> Primary Converter Full Bridge/2(G2)
  [G3] -> Primary Converter Full Bridge/3(G3)
  [G4] -> Primary Converter Full Bridge/4(G4)
  connections:
  Iin/LConn1 -- +/RConn1
  Vin/LConn1 -- Iin/RConn1 -- Primary Converter Full Bridge/LConn1
  Vin/RConn1 -- -/RConn1 -- Primary Converter Full Bridge/LConn2
  Primary Converter Full Bridge/RConn1 -- P/RConn1
  Primary Converter Full Bridge/RConn2 -- N/RConn1

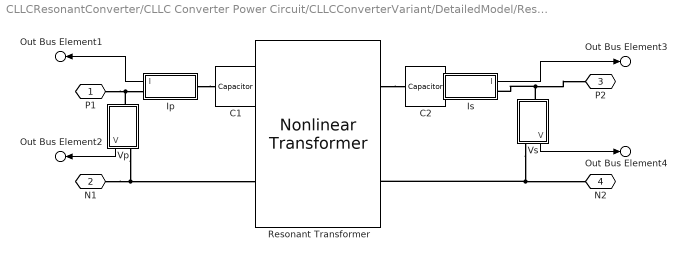
== system CLLCResonantConverter/CLLC Converter Power Circuit/CLLCConverterVariant/DetailedModel/Resonant Tank ==
  C1 : fl_lib/Electrical/Electrical Elements/Capacitor  c=C1 F  r=Rcr1 Ohm  g=0 1/Ohm  i_specify=off  i_priority=None  i=0 A  i_nominal_specify=off  i_nominal_value=1  i_nominal_unit=A  v_specify=off  v_priority=None  v=0 V  v_nominal_specify=off  v_nominal_value=1  v_nominal_unit=V  vc_specify=off  vc_priority=None  vc=0 V  vc_nominal_specify=off  vc_nominal_value=1  vc_nominal_unit=V
  C2 : fl_lib/Electrical/Electrical Elements/Capacitor  c=C2 F  r=Rcr2 Ohm  g=0 1/Ohm  i_specify=off  i_priority=None  i=0 A  i_nominal_specify=off  i_nominal_value=1  i_nominal_unit=A  v_specify=off  v_priority=None  v=0 V  v_nominal_specify=off  v_nominal_value=1  v_nominal_unit=V  vc_specify=off  vc_priority=None  vc=0 V  vc_nominal_specify=off  vc_nominal_value=1  vc_nominal_unit=V
  Ip : Subsystem
      settings: PortSchema="{\"entries\":[{\"content\":{\"sides\":[{\"content\":{\"connectorIds\":[\"Out1\",\"LConn1\"]},\"type\":\"ConnectorPlacement.EquallySpacedRectSide\",\"uuid\":\"e749c2ff-fd60-426f-a769-b61a7dfe80d2\"},{\"content\":{\"connectorIds\":[\"RConn1\"],\"side\":\"RIGHT\"},\"type\":\"ConnectorPlacement.EquallySpacedRectSide\",\"uuid\":\"f3bb02bd-f8d2-4326-b68c-6f969fa4ac22\"},{\"content\":{\"side\":\"TOP\"},\"type\":\"ConnectorPlacement.EquallySpacedRectSide\",\"uuid\":\"9ab7a0d1-20d8-49e4-8eb3-54d34434204c\"}]},\"type\":\"ConnectorPlacement.EquallySpacedConnector\",\"uuid\":\"19e2a6d5-13f4-47de-bb59-b826817cba83\"}],\"packageUris\":[\"http://schema.mathworks.com/mf0/Connector/R2020b\"],\"version\":\"1.0\"}"
      mask Display: disp("I")
  Is : Subsystem
      settings: PortSchema="{\"entries\":[{\"content\":{\"sides\":[{\"content\":{\"connectorIds\":[\"LConn1\"]},\"type\":\"ConnectorPlacement.EquallySpacedRectSide\",\"uuid\":\"e749c2ff-fd60-426f-a769-b61a7dfe80d2\"},{\"content\":{\"connectorIds\":[\"RConn1\",\"Out1\"],\"side\":\"RIGHT\"},\"type\":\"ConnectorPlacement.EquallySpacedRectSide\",\"uuid\":\"f3bb02bd-f8d2-4326-b68c-6f969fa4ac22\"},{\"content\":{\"side\":\"TOP\"},\"type\":\"ConnectorPlacement.EquallySpacedRectSide\",\"uuid\":\"9ab7a0d1-20d8-49e4-8eb3-54d34434204c\"}]},\"type\":\"ConnectorPlacement.EquallySpacedConnector\",\"uuid\":\"19e2a6d5-13f4-47de-bb59-b826817cba83\"}],\"packageUris\":[\"http://schema.mathworks.com/mf0/Connector/R2020b\"],\"version\":\"1.0\"}"
      mask Display: disp("I")
  Resonant Transformer : ee_lib/Passive/Transformers/Nonlinear Transformer  Nw=N1  Nw2=N2  winding_param_option=2  Req=0.01 Ohm  Leq=0.0001 H  R_1=R1 Ohm  L_1=Llk1 H  R_2=R2 Ohm  L_2=Llk2 H  averaging_period=0 s  R_m=10000 Ohm  parameterization_option=1  H_data=[0, 200, 400, 600, 800, 1000] A/m  B_data=[0, .81, 1.25, 1.42, 1.48, 1.49] T  length_effective=0.2 m  area_effective=2e-4 m^2  L=Lm H  L_sat=1e-2 H  current_data=[0, .4, .8, 1.2, 1.6, 2] A  magnetic_flux_data=[0, .161, .25, .284, .295, .299] .* 1e-3 Wb  magnetic_flux_sat=1.6e-04 Wb  dBdH0=0.005 T*m/A  B1=1.49 T  H1=1000 A/m  c=0.1  K=200 A/m  alpha=1e-4  interpolation_option=1  Leq_i0=0 A  L1_i0=0 A  L2_i0=0 A  x0_option=1  i_L0=0 A  phi0=0 Wb  B0=0 T  H0=0 A/m  Leq_g=1e-9 1/Ohm  L1_g=0 1/Ohm  L2_g=0 1/Ohm
  Vp : Subsystem
      mask Display: disp("V")
  Vs : Subsystem
      mask Display: disp("V")
  P1 : PMIOPort  Side=Left
  N1 : PMIOPort  Port=2  Side=Left
  P2 : PMIOPort  Port=3  Side=Right
  N2 : PMIOPort  Port=4  Side=Right
  Out Bus Element1 : Outport  PortName=meas  Element=Ip [A]
  Out Bus Element2 : Outport  PortName=meas  Element=Vp [V]
  Out Bus Element3 : Outport  PortName=meas  Element=Is [A]
  Out Bus Element4 : Outport  PortName=meas  Element=Vs [A]
  wires:
  Is/1(I) -> Out Bus Element3/1
  Vp/1(V) -> Out Bus Element2/1
  Ip/1(I) -> Out Bus Element1/1
  Vs/1(V) -> Out Bus Element4/1
  connections:
  C2/RConn1 -- Is/LConn1
  Resonant Transformer/RConn1 -- C2/LConn1
  Resonant Transformer/LConn1 -- C1/RConn1
  Ip/RConn1 -- C1/LConn1
  Vp/RConn1 -- N1/RConn1 -- Resonant Transformer/LConn2
  Vs/RConn1 -- Resonant Transformer/RConn2 -- N2/RConn1
  Vs/LConn1 -- Is/RConn1 -- P2/RConn1
  P1/RConn1 -- Vp/LConn1 -- Ip/LConn1

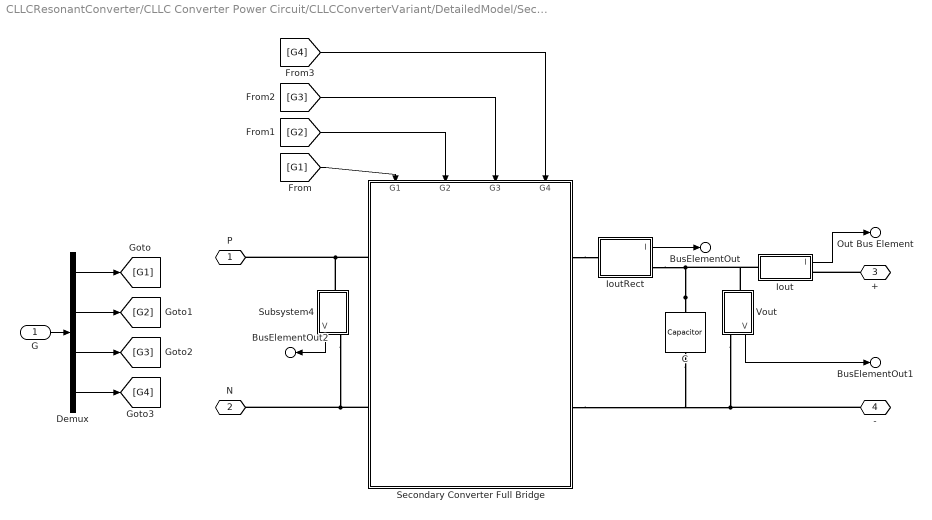
== system CLLCResonantConverter/CLLC Converter Power Circuit/CLLCConverterVariant/DetailedModel/Secondary Converter ==
  G : Inport
  C : fl_lib/Electrical/Electrical Elements/Capacitor  c=Co F  r=Rco Ohm  g=0 1/Ohm  i_specify=off  i_priority=None  i=0 A  i_nominal_specify=off  i_nominal_value=1  i_nominal_unit=A  v_specify=off  v_priority=None  v=450 V  v_nominal_specify=off  v_nominal_value=1  v_nominal_unit=V  vc_specify=on  vc_priority=High  vc=Vco V  vc_nominal_specify=off  vc_nominal_value=1  vc_nominal_unit=V
  Demux : Demux
  Iout : Subsystem
      mask Display: disp("I")
  IoutRect : Subsystem
      mask Display: disp("I")
  Secondary Converter Full Bridge : Subsystem  Variant=on  VariantControlMode=label  LabelModeActiveChoice=IdealMOSFETwithThermal
      settings: PortSchema="{\"entries\":[{\"content\":{\"sides\":[{\"content\":{\"connectorIds\":[\"LConn1\",\"LConn2\"]},\"type\":\"ConnectorPlacement.EquallySpacedRectSide\",\"uuid\":\"27c41940-d662-4779-afdd-48b642f77411\"},{\"content\":{\"connectorIds\":[\"RConn1\",\"RConn2\"],\"side\":\"RIGHT\"},\"type\":\"ConnectorPlacement.EquallySpacedRectSide\",\"uuid\":\"b0072b01-add1-4b0f-b94e-e1b6c9886b0e\"},{\"content\":{\"connectorIds\":[\"In1\",\"In2\",\"In3\",\"In4\"],\"side\":\"TOP\"},\"type\":\"ConnectorPlacement.EquallySpacedRectSide\",\"uuid\":\"c43bed80-422d-49db-9596-8b38d5c3e411\"},{\"content\":{\"side\":\"BOTTOM\"},\"type\":\"ConnectorPlacement.EquallySpacedRectSide\",\"uuid\":\"01f06046-f57e-45b0-bca5-368a5a543f97\"}]},\"type\":\"ConnectorPlacement.EquallySpacedConnector\",\"uuid\":\"2fcb5370-6bd7-4702-bf87-ebedbb7e376c\"}],\"packageUris\":[\"http://schema.mathworks.com/mf0/Connector/R2020b\"],\"version\":\"1.0\"}"
  Subsystem4 : Subsystem
      settings: PortSchema="{\"entries\":[{\"content\":{\"sides\":[{\"content\":{\"connectorIds\":[\"LConn1\"]},\"type\":\"ConnectorPlacement.EquallySpacedRectSide\",\"uuid\":\"e749c2ff-fd60-426f-a769-b61a7dfe80d2\"},{\"content\":{\"connectorIds\":[\"RConn1\",\"Out1\"],\"side\":\"RIGHT\"},\"type\":\"ConnectorPlacement.EquallySpacedRectSide\",\"uuid\":\"f3bb02bd-f8d2-4326-b68c-6f969fa4ac22\"},{\"content\":{\"side\":\"TOP\"},\"type\":\"ConnectorPlacement.EquallySpacedRectSide\",\"uuid\":\"9ab7a0d1-20d8-49e4-8eb3-54d34434204c\"}]},\"type\":\"ConnectorPlacement.EquallySpacedConnector\",\"uuid\":\"19e2a6d5-13f4-47de-bb59-b826817cba83\"}],\"packageUris\":[\"http://schema.mathworks.com/mf0/Connector/R2020b\"],\"version\":\"1.0\"}"
      mask Display: disp("V")
  Vout : Subsystem
      settings: PortSchema="{\"entries\":[{\"content\":{\"sides\":[{\"content\":{\"connectorIds\":[\"LConn1\"]},\"type\":\"ConnectorPlacement.EquallySpacedRectSide\",\"uuid\":\"e749c2ff-fd60-426f-a769-b61a7dfe80d2\"},{\"content\":{\"connectorIds\":[\"RConn1\",\"Out1\"],\"side\":\"RIGHT\"},\"type\":\"ConnectorPlacement.EquallySpacedRectSide\",\"uuid\":\"f3bb02bd-f8d2-4326-b68c-6f969fa4ac22\"},{\"content\":{\"side\":\"TOP\"},\"type\":\"ConnectorPlacement.EquallySpacedRectSide\",\"uuid\":\"9ab7a0d1-20d8-49e4-8eb3-54d34434204c\"}]},\"type\":\"ConnectorPlacement.EquallySpacedConnector\",\"uuid\":\"19e2a6d5-13f4-47de-bb59-b826817cba83\"}],\"packageUris\":[\"http://schema.mathworks.com/mf0/Connector/R2020b\"],\"version\":\"1.0\"}"
      mask Display: disp("V")
  P : PMIOPort  Side=Left
  N : PMIOPort  Port=2  Side=Left
  + : PMIOPort  Port=3  Side=Right
  - : PMIOPort  Port=4  Side=Right
  Out Bus Element : Outport  PortName=meas  Element=Iout [A]
  BusElementOut : Outport  PortName=meas  Element=IL [A]
  BusElementOut1 : Outport  PortName=meas  Element=Vout [V]
  BusElementOut2 : Outport  PortName=meas  Element=Vac [V]
  wires:
  [G4] -> Secondary Converter Full Bridge/4(G4)
  [G1] -> Secondary Converter Full Bridge/1(G1)
  [G3] -> Secondary Converter Full Bridge/3(G3)
  [G2] -> Secondary Converter Full Bridge/2(G2)
  Demux/3 -> [G3]
  Demux/4 -> [G4]
  G/1 -> Demux/1
  Demux/1 -> [G1]
  Demux/2 -> [G2]
  Subsystem4/1(V) -> BusElementOut2/1
  Vout/1(V) -> BusElementOut1/1
  IoutRect/1(I) -> BusElementOut/1
  Iout/1(I) -> Out Bus Element/1
  connections:
  +/RConn1 -- Iout/RConn1
  C/LConn1 -- Vout/LConn1 -- Iout/LConn1 -- IoutRect/RConn1
  -/RConn1 -- Secondary Converter Full Bridge/RConn2 -- C/RConn1 -- Vout/RConn1
  Subsystem4/LConn1 -- Secondary Converter Full Bridge/LConn1 -- P/RConn1
  Subsystem4/RConn1 -- Secondary Converter Full Bridge/LConn2 -- N/RConn1
  Secondary Converter Full Bridge/RConn1 -- IoutRect/LConn1

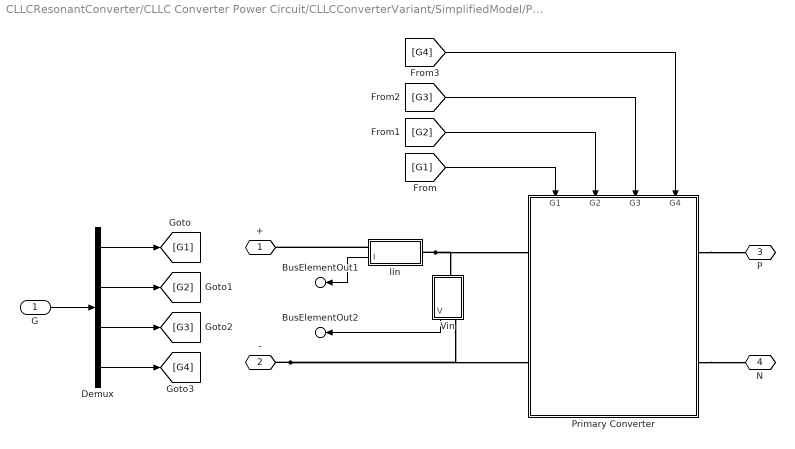
== system CLLCResonantConverter/CLLC Converter Power Circuit/CLLCConverterVariant/SimplifiedModel/Primary Converter ==
  G : Inport
  Demux : Demux
  Iin : Subsystem
      settings: PortSchema="{\"entries\":[{\"content\":{\"sides\":[{\"content\":{\"connectorIds\":[\"LConn1\",\"Out1\"]},\"type\":\"ConnectorPlacement.EquallySpacedRectSide\",\"uuid\":\"e749c2ff-fd60-426f-a769-b61a7dfe80d2\"},{\"content\":{\"connectorIds\":[\"RConn1\"],\"side\":\"RIGHT\"},\"type\":\"ConnectorPlacement.EquallySpacedRectSide\",\"uuid\":\"f3bb02bd-f8d2-4326-b68c-6f969fa4ac22\"},{\"content\":{\"side\":\"TOP\"},\"type\":\"ConnectorPlacement.EquallySpacedRectSide\",\"uuid\":\"9ab7a0d1-20d8-49e4-8eb3-54d34434204c\"}]},\"type\":\"ConnectorPlacement.EquallySpacedConnector\",\"uuid\":\"19e2a6d5-13f4-47de-bb59-b826817cba83\"}],\"packageUris\":[\"http://schema.mathworks.com/mf0/Connector/R2020b\"],\"version\":\"1.0\"}"
      mask Display: disp("I")
  Primary Converter : Subsystem  VariantControl=IdealSwitch
      settings: PortSchema="{\"entries\":[{\"content\":{\"sides\":[{\"content\":{\"connectorIds\":[\"LConn1\",\"LConn2\"]},\"type\":\"ConnectorPlacement.EquallySpacedRectSide\",\"uuid\":\"27c41940-d662-4779-afdd-48b642f77411\"},{\"content\":{\"connectorIds\":[\"RConn1\",\"RConn2\"],\"side\":\"RIGHT\"},\"type\":\"ConnectorPlacement.EquallySpacedRectSide\",\"uuid\":\"b0072b01-add1-4b0f-b94e-e1b6c9886b0e\"},{\"content\":{\"connectorIds\":[\"In1\",\"In2\",\"In3\",\"In4\"],\"side\":\"TOP\"},\"type\":\"ConnectorPlacement.EquallySpacedRectSide\",\"uuid\":\"c43bed80-422d-49db-9596-8b38d5c3e411\"},{\"content\":{\"side\":\"BOTTOM\"},\"type\":\"ConnectorPlacement.EquallySpacedRectSide\",\"uuid\":\"01f06046-f57e-45b0-bca5-368a5a543f97\"}]},\"type\":\"ConnectorPlacement.EquallySpacedConnector\",\"uuid\":\"2fcb5370-6bd7-4702-bf87-ebedbb7e376c\"}],\"packageUris\":[\"http://schema.mathworks.com/mf0/Connector/R2020b\"],\"version\":\"1.0\"}"
  Vin : Subsystem
      mask Display: disp("V")
  + : PMIOPort  Side=Left
  - : PMIOPort  Port=2  Side=Left
  P : PMIOPort  Port=3  Side=Right
  N : PMIOPort  Port=4  Side=Right
  BusElementOut2 : Outport  PortName=meas  Element=Vin [V]
  BusElementOut1 : Outport  PortName=meas  Element=Iin [A]
  wires:
  [G4] -> Primary Converter/4(G4)
  [G3] -> Primary Converter/3(G3)
  [G2] -> Primary Converter/2(G2)
  [G1] -> Primary Converter/1(G1)
  G/1 -> Demux/1
  Demux/1 -> [G1]
  Demux/2 -> [G2]
  Demux/3 -> [G3]
  Demux/4 -> [G4]
  Vin/1(V) -> BusElementOut2/1
  Iin/1(I) -> BusElementOut1/1
  connections:
  Primary Converter/RConn2 -- N/RConn1
  Primary Converter/RConn1 -- P/RConn1
  -/RConn1 -- Primary Converter/LConn2 -- Vin/RConn1
  Iin/RConn1 -- Primary Converter/LConn1 -- Vin/LConn1
  Iin/LConn1 -- +/RConn1

== system CLLCResonantConverter/CLLC Converter Power Circuit/CLLCConverterVariant/SimplifiedModel/Resonant Tank ==
  C1 : fl_lib/Electrical/Electrical Elements/Capacitor  c=C1 F  r=Rcr1 Ohm  g=0 1/Ohm  i_specify=off  i_priority=None  i=0 A  i_nominal_specify=off  i_nominal_value=1  i_nominal_unit=A  v_specify=off  v_priority=None  v=0 V  v_nominal_specify=off  v_nominal_value=1  v_nominal_unit=V  vc_specify=off  vc_priority=None  vc=0 V  vc_nominal_specify=off  vc_nominal_value=1  vc_nominal_unit=V
  C2 : fl_lib/Electrical/Electrical Elements/Capacitor  c=C2 F  r=Rcr2 Ohm  g=0 1/Ohm  i_specify=off  i_priority=None  i=0 A  i_nominal_specify=off  i_nominal_value=1  i_nominal_unit=A  v_specify=off  v_priority=None  v=0 V  v_nominal_specify=off  v_nominal_value=1  v_nominal_unit=V  vc_specify=off  vc_priority=None  vc=0 V  vc_nominal_specify=off  vc_nominal_value=1  vc_nominal_unit=V
  Ip : Subsystem
      settings: PortSchema="{\"entries\":[{\"content\":{\"sides\":[{\"content\":{\"connectorIds\":[\"Out1\",\"LConn1\"]},\"type\":\"ConnectorPlacement.EquallySpacedRectSide\",\"uuid\":\"e749c2ff-fd60-426f-a769-b61a7dfe80d2\"},{\"content\":{\"connectorIds\":[\"RConn1\"],\"side\":\"RIGHT\"},\"type\":\"ConnectorPlacement.EquallySpacedRectSide\",\"uuid\":\"f3bb02bd-f8d2-4326-b68c-6f969fa4ac22\"},{\"content\":{\"side\":\"TOP\"},\"type\":\"ConnectorPlacement.EquallySpacedRectSide\",\"uuid\":\"9ab7a0d1-20d8-49e4-8eb3-54d34434204c\"}]},\"type\":\"ConnectorPlacement.EquallySpacedConnector\",\"uuid\":\"19e2a6d5-13f4-47de-bb59-b826817cba83\"}],\"packageUris\":[\"http://schema.mathworks.com/mf0/Connector/R2020b\"],\"version\":\"1.0\"}"
      mask Display: disp("I")
  Is : Subsystem
      settings: PortSchema="{\"entries\":[{\"content\":{\"sides\":[{\"content\":{\"connectorIds\":[\"LConn1\"]},\"type\":\"ConnectorPlacement.EquallySpacedRectSide\",\"uuid\":\"e749c2ff-fd60-426f-a769-b61a7dfe80d2\"},{\"content\":{\"connectorIds\":[\"RConn1\",\"Out1\"],\"side\":\"RIGHT\"},\"type\":\"ConnectorPlacement.EquallySpacedRectSide\",\"uuid\":\"f3bb02bd-f8d2-4326-b68c-6f969fa4ac22\"},{\"content\":{\"side\":\"TOP\"},\"type\":\"ConnectorPlacement.EquallySpacedRectSide\",\"uuid\":\"9ab7a0d1-20d8-49e4-8eb3-54d34434204c\"}]},\"type\":\"ConnectorPlacement.EquallySpacedConnector\",\"uuid\":\"19e2a6d5-13f4-47de-bb59-b826817cba83\"}],\"packageUris\":[\"http://schema.mathworks.com/mf0/Connector/R2020b\"],\"version\":\"1.0\"}"
      mask Display: disp("I")
  Resonant Transformer : ee_lib/Passive/Transformers/Mutual Inductor  L1=Lm+Llk1 H  L2=Lm/(N1/N2)^2+Llk2 H  k=Lm/sqrt((Lm+Llk1)*(Lm+(N1/N2)^2*Llk2))  L_tol=20  enable_L1_tol=ee.enum.toleranceApplication.none  L1_tol_distribution=ee.enum.toleranceDistribution.uniform  L1_nSigma=4  enable_L2_tol=ee.enum.toleranceApplication.none  L2_tol_distribution=ee.enum.toleranceDistribution.uniform  L2_nSigma=4  r=[R1, R2] Ohm  g=[1e-09, 1e-09] 1/Ohm  enable_operating_limits=ee.enum.enable.no  operating_limit_action=ee.enum.passive.reportOpLim.warn  max_working_current=1 A  power_rating=1 W  iL1_specify=off  iL1_priority=High  iL1=0 A  iL1_nominal_specify=off  iL1_nominal_value=1  iL1_nominal_unit=A  iL2_specify=off  iL2_priority=High  iL2=0 A  iL2_nominal_specify=off  iL2_nominal_value=1  iL2_nominal_unit=A
  Vp : Subsystem
      mask Display: disp("V")
  Vs : Subsystem
      mask Display: disp("V")
  P1 : PMIOPort  Side=Left
  N1 : PMIOPort  Port=2  Side=Left
  P2 : PMIOPort  Port=3  Side=Right
  N2 : PMIOPort  Port=4  Side=Right
  Out Bus Element1 : Outport  PortName=meas  Element=Ip [A]
  Out Bus Element2 : Outport  PortName=meas  Element=Vp [V]
  Out Bus Element3 : Outport  PortName=meas  Element=Is [A]
  Out Bus Element4 : Outport  PortName=meas  Element=Vs [A]
  wires:
  Vs/1(V) -> Out Bus Element4/1
  Ip/1(I) -> Out Bus Element1/1
  Vp/1(V) -> Out Bus Element2/1
  Is/1(I) -> Out Bus Element3/1
  connections:
  Ip/LConn1 -- Vp/LConn1 -- P1/RConn1
  P2/RConn1 -- Is/RConn1 -- Vs/LConn1
  N2/RConn1 -- Resonant Transformer/RConn2 -- Vs/RConn1
  Resonant Transformer/LConn2 -- N1/RConn1 -- Vp/RConn1
  Ip/RConn1 -- C1/LConn1
  Resonant Transformer/LConn1 -- C1/RConn1
  Resonant Transformer/RConn1 -- C2/LConn1
  C2/RConn1 -- Is/LConn1
